simulink model "MOBATSim"  (R2020b)
settings: Solver=FixedStepAuto  StartTime=0.0  StopTime=Sim_t  FixedStep=0.01  MinStep=0.01  RelTol=1e-2
values from neighbouring files (symbols this model uses):
  Vehicles = evalin('base','Vehicles')    [I2V.m]    (also in VehicleSensors.m)
undefined symbols (not defined in the file or in its folder): Sim_Ts
libraries: simulink x50, robotalgslib x10, drivingvehiclecontroller x10, mpcadaslib x10, pid_lib x10
(part 1 of 7)
Description:
  | Main Simulink Model for MOBATSim
settings Model: VariantFading=off  Creator=Mustafa  LastModifiedBy=mustafa
settings SolverCC: AutoInsertRateTranBlk=on  InsertRTBMode=Always  MinimalZcImpactIntegration=on
settings DataIOCC: ReturnWorkspaceOutputs=off
settings DebuggingCC: AlgebraicLoopMsg=error  UniqueDataStoreMsg=error  ArithmeticOperatorsInVariantConditions=warning
settings SFSimCC: SimUseLocalCustomCode=off  CustomCodeUndefinedFunction=UseInterfaceOnly
settings RTWCC: RTWUseLocalCustomCode=off
settings CodeAppCC: StateflowObjectComments=on

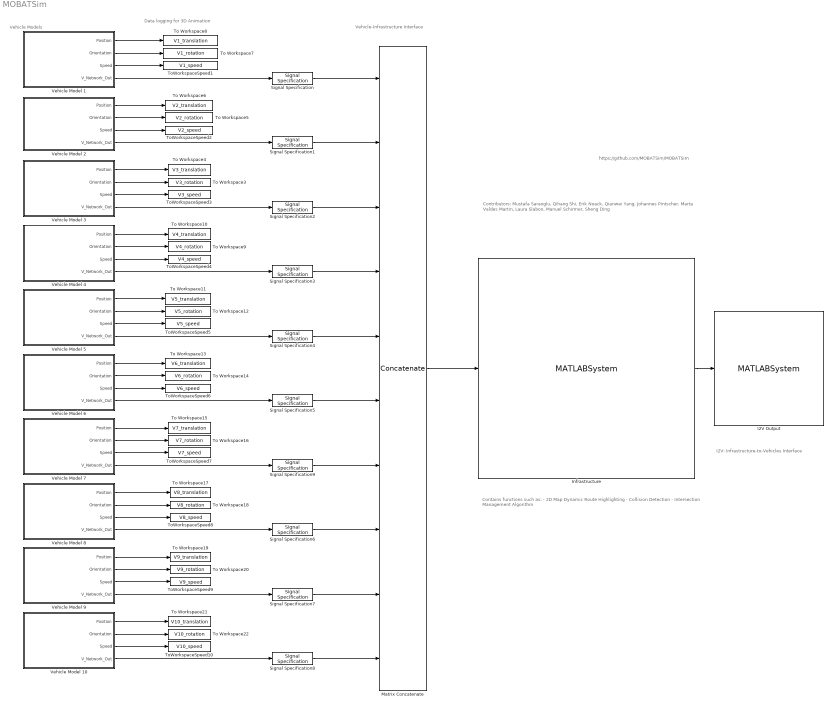
== system MOBATSim ==
  note: Contributors: Mustafa Saraoglu, Qihang Shi, Erik Noack, Qianwei Yang, Johannes Pintscher, Marta Valdes Martin, Laura Slabon, Manuel Schirmer, Sheng Ding
  note: https://github.com/MOBATSim/MOBATSim
  note: Data logging for 3D Animation
  note: Vehicle Models
  note: Vehicle-Infrastructure Interface
  note: I2V: Infrastructure-to-Vehicles Interface
  note: Contains functions such as:
      | - 2D Map Dynamic Route Highlighting
      | - Collision Detection
      | - Intersection Management Algorithm
  I2V Output : MATLABSystem  System=I2V  SimulateUsing=Interpreted execution
      mask Type: I2V
      mask Display:
      | image('MOBATSIM-Icon-Set_3- Flags.png');
      | port_label('input',1,'Flags');
  Infrastructure : MATLABSystem  Description=An instance of the Map.m Class is created.  System=Infrastructure  nrVehicles=length(Vehicles)  SimulateUsing=Interpreted execution
      mask Type: Infrastructure
      mask Display:
      | image('MOBATSIM-Icon-Set_5- Intersection.png');
      | port_label('input',1,'V2Idata');
      | port_label('output',1,'StopCommands');
  Matrix Concatenate : Concatenate  NumInputs=10  Mode=Multidimensional array
  Signal Specification{,1..9} (10 alike) : SignalSpecification  Dimensions=[1 2]
  To Workspace10 : ToWorkspace  VariableName=V4_translation  SaveFormat=Timeseries  SampleTime=-1
  To Workspace11 : ToWorkspace  VariableName=V5_translation  SaveFormat=Timeseries  SampleTime=-1
  To Workspace12 : ToWorkspace  VariableName=V5_rotation  SaveFormat=Timeseries  SampleTime=-1
  To Workspace13 : ToWorkspace  VariableName=V6_translation  SaveFormat=Timeseries  SampleTime=-1
  To Workspace14 : ToWorkspace  VariableName=V6_rotation  SaveFormat=Timeseries  SampleTime=-1
  To Workspace15 : ToWorkspace  VariableName=V7_translation  SaveFormat=Timeseries  SampleTime=-1
  To Workspace16 : ToWorkspace  VariableName=V7_rotation  SaveFormat=Timeseries  SampleTime=-1
  To Workspace17 : ToWorkspace  VariableName=V8_translation  SaveFormat=Timeseries  SampleTime=-1
  To Workspace18 : ToWorkspace  VariableName=V8_rotation  SaveFormat=Timeseries  SampleTime=-1
  To Workspace19 : ToWorkspace  VariableName=V9_translation  SaveFormat=Timeseries  SampleTime=-1
  To Workspace20 : ToWorkspace  VariableName=V9_rotation  SaveFormat=Timeseries  SampleTime=-1
  To Workspace21 : ToWorkspace  VariableName=V10_translation  SaveFormat=Timeseries  SampleTime=-1
  To Workspace22 : ToWorkspace  VariableName=V10_rotation  SaveFormat=Timeseries  SampleTime=-1
  To Workspace3 : ToWorkspace  VariableName=V3_rotation  SaveFormat=Timeseries  SampleTime=-1
  To Workspace4 : ToWorkspace  VariableName=V3_translation  SaveFormat=Timeseries  SampleTime=-1
  To Workspace5 : ToWorkspace  VariableName=V2_rotation  SaveFormat=Timeseries  SampleTime=-1
  To Workspace6 : ToWorkspace  VariableName=V2_translation  SaveFormat=Timeseries  SampleTime=-1
  To Workspace7 : ToWorkspace  VariableName=V1_rotation  SaveFormat=Timeseries  SampleTime=-1
  To Workspace8 : ToWorkspace  VariableName=V1_translation  SaveFormat=Timeseries  SampleTime=-1
  To Workspace9 : ToWorkspace  VariableName=V4_rotation  SaveFormat=Timeseries  SampleTime=-1
  ToWorkspaceSpeed1 : ToWorkspace  VariableName=V1_speed  SaveFormat=Timeseries  SampleTime=-1
  ToWorkspaceSpeed10 : ToWorkspace  VariableName=V10_speed  SaveFormat=Timeseries  SampleTime=-1
  ToWorkspaceSpeed2 : ToWorkspace  VariableName=V2_speed  SaveFormat=Timeseries  SampleTime=-1
  "ToWorkspaceSpeed3 " : ToWorkspace  VariableName=V3_speed  SaveFormat=Timeseries  SampleTime=-1
  ToWorkspaceSpeed4 : ToWorkspace  VariableName=V4_speed  SaveFormat=Timeseries  SampleTime=-1
  ToWorkspaceSpeed5 : ToWorkspace  VariableName=V5_speed  SaveFormat=Timeseries  SampleTime=-1
  ToWorkspaceSpeed6 : ToWorkspace  VariableName=V6_speed  SaveFormat=Timeseries  SampleTime=-1
  ToWorkspaceSpeed7 : ToWorkspace  VariableName=V7_speed  SaveFormat=Timeseries  SampleTime=-1
  ToWorkspaceSpeed8 : ToWorkspace  VariableName=V8_speed  SaveFormat=Timeseries  SampleTime=-1
  ToWorkspaceSpeed9 : ToWorkspace  VariableName=V9_speed  SaveFormat=Timeseries  SampleTime=-1
  Vehicle Model 1 : Subsystem  Description=Tag: Autonomous Vehicle Model  SystemSampleTime=0.01  mask{Vehicle_id=1}
      mask TypeOptions Vehicle_id: MATLAB System2/Vehicle_id
      mask DialogControl DescTextVar Prompt: Autonomous Vehicle Model defined as a system, press the arrow on the lower left corner to see the subsystems. The initial parameters below should be taken from the base workspace but you can edit them anyway you like.
      mask Display: image('$imagefile'); % Use "Edit Image" on toolstrip to change.
  Vehicle Model 10 : Subsystem  Description=Tag: Autonomous Vehicle Model  SystemSampleTime=0.01  mask{Vehicle_id=10}
      mask TypeOptions Vehicle_id: MATLAB System2/Vehicle_id
      mask DialogControl DescTextVar Prompt: Autonomous Vehicle Model defined as a system, press the arrow on the lower left corner to see the subsystems. The initial parameters below should be taken from the base workspace but you can edit them anyway you like.
      mask Display: image('$imagefile'); % Use "Edit Image" on toolstrip to change.
  Vehicle Model 2 : Subsystem  Description=Tag: Autonomous Vehicle Model  SystemSampleTime=0.01  mask{Vehicle_id=2}
      mask TypeOptions Vehicle_id: MATLAB System2/Vehicle_id
      mask DialogControl DescTextVar Prompt: Autonomous Vehicle Model defined as a system, press the arrow on the lower left corner to see the subsystems. The initial parameters below should be taken from the base workspace but you can edit them anyway you like.
      mask Display: image('$imagefile'); % Use "Edit Image" on toolstrip to change.
  Vehicle Model 3 : Subsystem  Description=Tag: Autonomous Vehicle Model  SystemSampleTime=0.01  mask{Vehicle_id=3}
      mask TypeOptions Vehicle_id: MATLAB System2/Vehicle_id
      mask DialogControl DescTextVar Prompt: Autonomous Vehicle Model defined as a system, press the arrow on the lower left corner to see the subsystems. The initial parameters below should be taken from the base workspace but you can edit them anyway you like.
      mask Display: image('$imagefile'); % Use "Edit Image" on toolstrip to change.
  Vehicle Model 4 : Subsystem  Description=Tag: Autonomous Vehicle Model  SystemSampleTime=0.01  mask{Vehicle_id=4}
      mask TypeOptions Vehicle_id: MATLAB System2/Vehicle_id
      mask DialogControl DescTextVar Prompt: Autonomous Vehicle Model defined as a system, press the arrow on the lower left corner to see the subsystems. The initial parameters below should be taken from the base workspace but you can edit them anyway you like.
      mask Display: image('$imagefile'); % Use "Edit Image" on toolstrip to change.
  Vehicle Model 5 : Subsystem  Description=Tag: Autonomous Vehicle Model  SystemSampleTime=0.01  mask{Vehicle_id=5}
      mask TypeOptions Vehicle_id: MATLAB System2/Vehicle_id
      mask DialogControl DescTextVar Prompt: Autonomous Vehicle Model defined as a system, press the arrow on the lower left corner to see the subsystems. The initial parameters below should be taken from the base workspace but you can edit them anyway you like.
      mask Display: image('$imagefile'); % Use "Edit Image" on toolstrip to change.
  Vehicle Model 6 : Subsystem  Description=Tag: Autonomous Vehicle Model  SystemSampleTime=0.01  mask{Vehicle_id=6}
      mask TypeOptions Vehicle_id: MATLAB System2/Vehicle_id
      mask DialogControl DescTextVar Prompt: Autonomous Vehicle Model defined as a system, press the arrow on the lower left corner to see the subsystems. The initial parameters below should be taken from the base workspace but you can edit them anyway you like.
      mask Display: image('$imagefile'); % Use "Edit Image" on toolstrip to change.
  Vehicle Model 7 : Subsystem  Description=Tag: Autonomous Vehicle Model  SystemSampleTime=0.01  mask{Vehicle_id=7}
      mask TypeOptions Vehicle_id: MATLAB System2/Vehicle_id
      mask DialogControl DescTextVar Prompt: Autonomous Vehicle Model defined as a system, press the arrow on the lower left corner to see the subsystems. The initial parameters below should be taken from the base workspace but you can edit them anyway you like.
      mask Display: image('$imagefile'); % Use "Edit Image" on toolstrip to change.
  Vehicle Model 8 : Subsystem  Description=Tag: Autonomous Vehicle Model  SystemSampleTime=0.01  mask{Vehicle_id=8}
      mask TypeOptions Vehicle_id: MATLAB System2/Vehicle_id
      mask DialogControl DescTextVar Prompt: Autonomous Vehicle Model defined as a system, press the arrow on the lower left corner to see the subsystems. The initial parameters below should be taken from the base workspace but you can edit them anyway you like.
      mask Display: image('$imagefile'); % Use "Edit Image" on toolstrip to change.
  Vehicle Model 9 : Subsystem  Description=Tag: Autonomous Vehicle Model  SystemSampleTime=0.01  mask{Vehicle_id=9}
      mask TypeOptions Vehicle_id: MATLAB System2/Vehicle_id
      mask DialogControl DescTextVar Prompt: Autonomous Vehicle Model defined as a system, press the arrow on the lower left corner to see the subsystems. The initial parameters below should be taken from the base workspace but you can edit them anyway you like.
      mask Display: image('$imagefile'); % Use "Edit Image" on toolstrip to change.
  wires:
  Vehicle Model 1/1(Position) -> To Workspace8/1
  Vehicle Model 1/2(Orientation) -> To Workspace7/1
  Vehicle Model 1/4(V_Network_Out) -> Signal Specification/1
  Signal Specification/1 -> Matrix Concatenate/1
  Signal Specification1/1 -> Matrix Concatenate/2
  Vehicle Model 2/2(Orientation) -> To Workspace5/1
  Vehicle Model 2/1(Position) -> To Workspace6/1
  Vehicle Model 3/2(Orientation) -> To Workspace3/1
  Vehicle Model 3/1(Position) -> To Workspace4/1
  Signal Specification2/1 -> Matrix Concatenate/3
  Infrastructure/1 -> I2V Output/1
  Vehicle Model 8/4(V_Network_Out) -> Signal Specification6/1
  Vehicle Model 9/4(V_Network_Out) -> Signal Specification7/1
  Vehicle Model 10/4(V_Network_Out) -> Signal Specification8/1
  Signal Specification3/1 -> Matrix Concatenate/4
  Signal Specification4/1 -> Matrix Concatenate/5
  Signal Specification5/1 -> Matrix Concatenate/6
  Signal Specification9/1 -> Matrix Concatenate/7
  Signal Specification6/1 -> Matrix Concatenate/8
  Signal Specification7/1 -> Matrix Concatenate/9
  Signal Specification8/1 -> Matrix Concatenate/10
  Vehicle Model 4/2(Orientation) -> To Workspace9/1
  Vehicle Model 4/1(Position) -> To Workspace10/1
  Vehicle Model 6/2(Orientation) -> To Workspace14/1
  Vehicle Model 6/1(Position) -> To Workspace13/1
  Vehicle Model 7/2(Orientation) -> To Workspace16/1
  Vehicle Model 7/1(Position) -> To Workspace15/1
  Vehicle Model 8/2(Orientation) -> To Workspace18/1
  Vehicle Model 8/1(Position) -> To Workspace17/1
  Vehicle Model 9/2(Orientation) -> To Workspace20/1
  Vehicle Model 9/1(Position) -> To Workspace19/1
  Vehicle Model 10/2(Orientation) -> To Workspace22/1
  Vehicle Model 10/1(Position) -> To Workspace21/1
  Matrix Concatenate/1 -> Infrastructure/1
  Vehicle Model 2/4(V_Network_Out) -> Signal Specification1/1
  Vehicle Model 3/4(V_Network_Out) -> Signal Specification2/1
  Vehicle Model 4/4(V_Network_Out) -> Signal Specification3/1
  Vehicle Model 6/4(V_Network_Out) -> Signal Specification5/1
  Vehicle Model 7/4(V_Network_Out) -> Signal Specification9/1
  Vehicle Model 5/1(Position) -> To Workspace11/1
  Vehicle Model 5/2(Orientation) -> To Workspace12/1
  Vehicle Model 5/4(V_Network_Out) -> Signal Specification4/1
  Vehicle Model 1/3(Speed) -> ToWorkspaceSpeed1/1
  Vehicle Model 2/3(Speed) -> ToWorkspaceSpeed2/1
  Vehicle Model 3/3(Speed) -> "ToWorkspaceSpeed3 "/1
  Vehicle Model 4/3(Speed) -> ToWorkspaceSpeed4/1
  Vehicle Model 5/3(Speed) -> ToWorkspaceSpeed5/1
  Vehicle Model 6/3(Speed) -> ToWorkspaceSpeed6/1
  Vehicle Model 7/3(Speed) -> ToWorkspaceSpeed7/1
  Vehicle Model 8/3(Speed) -> ToWorkspaceSpeed8/1
  Vehicle Model 9/3(Speed) -> ToWorkspaceSpeed9/1
  Vehicle Model 10/3(Speed) -> ToWorkspaceSpeed10/1

== system MOBATSim/Vehicle Model 1 ==
  note: Perception
  note: Decision-Making
  note: Control
  Behavioural Planner : MATLABSystem  System=VehicleDrivingMode  Vehicle_id=Vehicle_id  SimulateUsing=Interpreted execution
      mask Type: VehicleDrivingMode
      mask Display:
      | image('MOBATSIM-Icon-Set_7- Behavioural Planner.png');
      | port_label('input',1,'vehicleDetected');
      | port_label('output',1,'SpeedReference');
      | port_label('output',2,'DistanceReference');
      | port_label('output',3,'LeadSpeed');
      | port_label('output',4,'DrivingMode');
      | port_label('output',5,'Dist2Stop');
      | port_label('output',6,'laneChange');
  Longitudinal and Lateral Controllers : Subsystem
  Path Planner : Subsystem  Variant=on  VariantControlMode=label  LabelModeActiveChoice=Astar  mask{PathPlanningAlgorithm=Astar}
      mask prompts: PathPlanningAlgorithm "Path Planning Algorithm"
      mask TypeOptions PathPlanningAlgorithm: Astar | ShortestPathFinder
      mask Callback PathPlanningAlgorithm: set_param(gcb,'OverrideUsingVariant',get_param(gcb,'PathPlanningAlgorithm'));
      mask Display: image("MOBATSIM-Icon-Set_8- Navigation.png");
  Transform to MOBATSim Coordinates : Subsystem
  Vehicle Model : Subsystem  mask{Vehicle_id=Vehicle_id}
      mask prompts: Vehicle_id "Vehicle ID"
      mask Display: image('MOBATSIM-Icon-Set_13- VehicleModel.png'); % Use "Edit Image" on toolstrip to change.
  Vehicle Sensors : MATLABSystem  System=VehicleSensors  Vehicle_id=Vehicle_id  Tsample=Sim_Ts  OffsetTime=0  SimulateUsing=Interpreted execution
      mask Type: VehicleSensors
      mask Display:
      | image('MOBATSIM-Icon-Set_4- Sensor.png');
      | port_label('output',1,'V2VcommIDs');
      | port_label('output',2,'vehicleDetected');
  Vehicle Status Check and Acceleration to Speed : Subsystem
  Vehicle V2I Output : MATLABSystem  System=VehicleV2I_Out  Vehicle_id=Vehicle_id  SimulateUsing=Interpreted execution
      mask Type: VehicleV2I_Out
      mask Display:
      | image('MOBATSIM-Icon-Set_6- V2l.png');
      | port_label('input',1,'waypointReached');
      | port_label('output',1,'V2Idata');
  Position : Outport  VectorParamsAs1DForOutWhenUnconnected=off
  Orientation : Outport  Port=2  VectorParamsAs1DForOutWhenUnconnected=off
  Speed : Outport  Port=3  VectorParamsAs1DForOutWhenUnconnected=off
  V_Network_Out : Outport  Port=4  VectorParamsAs1DForOutWhenUnconnected=off
  wires:
  Vehicle V2I Output/1 -> V_Network_Out/1
  Vehicle Sensors/2 -> Behavioural Planner/1
  Behavioural Planner/1 -> Longitudinal and Lateral Controllers/1(Speed Reference)
  Behavioural Planner/2 -> Longitudinal and Lateral Controllers/2(Inter Vehicular Distance)
  Behavioural Planner/3 -> Longitudinal and Lateral Controllers/3(Lead Speed)
  Behavioural Planner/4 -> Longitudinal and Lateral Controllers/4(drivingMode)
  Behavioural Planner/5 -> Longitudinal and Lateral Controllers/5(Dist2Stop)
  Transform to MOBATSim Coordinates/1(Position) -> Position/1
  Transform to MOBATSim Coordinates/2(Orientation) -> Orientation/1
  Vehicle Model/2(Speed) -> Longitudinal and Lateral Controllers/8(Actual Speed), Speed/1
  Vehicle Model/1(Pose) -> Longitudinal and Lateral Controllers/7(Actual Pose), Transform to MOBATSim Coordinates/1(Pose)
  Longitudinal and Lateral Controllers/1(Longitudinal Acceleration Cmd) -> Vehicle Status Check and Acceleration to Speed/1(Reference Acceleration)
  Longitudinal and Lateral Controllers/2(Reference Steering Angle) -> Vehicle Status Check and Acceleration to Speed/2(Reference Steering Angle)
  Vehicle Status Check and Acceleration to Speed/2(Steering Angle Cmd) -> Vehicle Model/2(Steering Angle)
  Behavioural Planner/6 -> Longitudinal and Lateral Controllers/6(laneChange)
  Vehicle Sensors/1 -> Path Planner/1(CommunicationIDs)
  Path Planner/1(waypointReached) -> Vehicle V2I Output/1
  Vehicle Status Check and Acceleration to Speed/1(Speed Cmd) -> Vehicle Model/1(Longitudinal Speed)

== system MOBATSim/Vehicle Model 10 ==
  note: Perception
  note: Decision-Making
  note: Control
  Behavioural Planner : MATLABSystem  System=VehicleDrivingMode  Vehicle_id=Vehicle_id  SimulateUsing=Interpreted execution
      mask Type: VehicleDrivingMode
      mask Display:
      | image('MOBATSIM-Icon-Set_7- Behavioural Planner.png');
      | port_label('input',1,'vehicleDetected');
      | port_label('output',1,'SpeedReference');
      | port_label('output',2,'DistanceReference');
      | port_label('output',3,'LeadSpeed');
      | port_label('output',4,'DrivingMode');
      | port_label('output',5,'Dist2Stop');
      | port_label('output',6,'laneChange');
  Longitudinal and Lateral Controllers : Subsystem
  Path Planner : Subsystem  Variant=on  VariantControlMode=label  LabelModeActiveChoice=Astar  mask{PathPlanningAlgorithm=Astar}
      mask prompts: PathPlanningAlgorithm "Path Planning Algorithm"
      mask TypeOptions PathPlanningAlgorithm: Astar | ShortestPathFinder
      mask Callback PathPlanningAlgorithm: set_param(gcb,'OverrideUsingVariant',get_param(gcb,'PathPlanningAlgorithm'));
      mask Display: image("MOBATSIM-Icon-Set_8- Navigation.png");
  Transform to MOBATSim Coordinates : Subsystem
  Vehicle Model : Subsystem  mask{Vehicle_id=Vehicle_id}
      mask prompts: Vehicle_id "Vehicle ID"
      mask Display: image('MOBATSIM-Icon-Set_13- VehicleModel.png'); % Use "Edit Image" on toolstrip to change.
  Vehicle Sensors : MATLABSystem  System=VehicleSensors  Vehicle_id=Vehicle_id  Tsample=Sim_Ts  OffsetTime=0  SimulateUsing=Interpreted execution
      mask Type: VehicleSensors
      mask Display:
      | image('MOBATSIM-Icon-Set_4- Sensor.png');
      | port_label('output',1,'V2VcommIDs');
      | port_label('output',2,'vehicleDetected');
  Vehicle Status Check and Acceleration to Speed : Subsystem
  Vehicle V2I Output : MATLABSystem  System=VehicleV2I_Out  Vehicle_id=Vehicle_id  SimulateUsing=Interpreted execution
      mask Type: VehicleV2I_Out
      mask Display:
      | image('MOBATSIM-Icon-Set_6- V2l.png');
      | port_label('input',1,'waypointReached');
      | port_label('output',1,'V2Idata');
  Position : Outport  VectorParamsAs1DForOutWhenUnconnected=off
  Orientation : Outport  Port=2  VectorParamsAs1DForOutWhenUnconnected=off
  Speed : Outport  Port=3  VectorParamsAs1DForOutWhenUnconnected=off
  V_Network_Out : Outport  Port=4  VectorParamsAs1DForOutWhenUnconnected=off
  wires:
  Vehicle V2I Output/1 -> V_Network_Out/1
  Vehicle Sensors/2 -> Behavioural Planner/1
  Behavioural Planner/1 -> Longitudinal and Lateral Controllers/1(Speed Reference)
  Behavioural Planner/2 -> Longitudinal and Lateral Controllers/2(Inter Vehicular Distance)
  Behavioural Planner/3 -> Longitudinal and Lateral Controllers/3(Lead Speed)
  Behavioural Planner/4 -> Longitudinal and Lateral Controllers/4(drivingMode)
  Behavioural Planner/5 -> Longitudinal and Lateral Controllers/5(Dist2Stop)
  Transform to MOBATSim Coordinates/1(Position) -> Position/1
  Transform to MOBATSim Coordinates/2(Orientation) -> Orientation/1
  Vehicle Model/2(Speed) -> Longitudinal and Lateral Controllers/8(Actual Speed), Speed/1
  Vehicle Model/1(Pose) -> Longitudinal and Lateral Controllers/7(Actual Pose), Transform to MOBATSim Coordinates/1(Pose)
  Longitudinal and Lateral Controllers/1(Longitudinal Acceleration Cmd) -> Vehicle Status Check and Acceleration to Speed/1(Reference Acceleration)
  Longitudinal and Lateral Controllers/2(Reference Steering Angle) -> Vehicle Status Check and Acceleration to Speed/2(Reference Steering Angle)
  Vehicle Status Check and Acceleration to Speed/2(Steering Angle Cmd) -> Vehicle Model/2(Steering Angle)
  Behavioural Planner/6 -> Longitudinal and Lateral Controllers/6(laneChange)
  Vehicle Sensors/1 -> Path Planner/1(CommunicationIDs)
  Path Planner/1(waypointReached) -> Vehicle V2I Output/1
  Vehicle Status Check and Acceleration to Speed/1(Speed Cmd) -> Vehicle Model/1(Longitudinal Speed)

== system MOBATSim/Vehicle Model 2 ==
  note: Decision-Making
  note: Control
  note: Perception
  note: Vehicle 2: Ego Vehicle in 3D
      | - Lane-changing on double-lane routes
  Behavioural Planner - Ego Vehicle : MATLABSystem  System=VehicleDrivingMode_Ego  Vehicle_id=Vehicle_id  SimulateUsing=Interpreted execution
      mask Type: VehicleDrivingMode_Ego
      mask Display:
      | image('MOBATSIM-Icon-Set_7- Behavioural Planner.png');
      | port_label('input',1,'vehicleDetected');
      | port_label('output',1,'SpeedReference');
      | port_label('output',2,'DistanceReference');
      | port_label('output',3,'LeadSpeed');
      | port_label('output',4,'DrivingMode');
      | port_label('output',5,'Dist2Stop');
      | port_label('output',6,'laneChange');
  Longitudinal and Lateral Controllers : Subsystem
  Path Planner : Subsystem  Variant=on  VariantControlMode=label  LabelModeActiveChoice=Astar  mask{PathPlanningAlgorithm=Astar}
      mask prompts: PathPlanningAlgorithm "Path Planning Algorithm"
      mask TypeOptions PathPlanningAlgorithm: Astar | ShortestPathFinder
      mask Callback PathPlanningAlgorithm: set_param(gcb,'OverrideUsingVariant',get_param(gcb,'PathPlanningAlgorithm'));
      mask Display: image("MOBATSIM-Icon-Set_8- Navigation.png");
  Transform to MOBATSim Coordinates : Subsystem
  Vehicle Model : Subsystem  mask{Vehicle_id=Vehicle_id}
      mask prompts: Vehicle_id "Vehicle ID"
      mask Display: image('MOBATSIM-Icon-Set_13- VehicleModel.png'); % Use "Edit Image" on toolstrip to change.
  Vehicle Sensors : MATLABSystem  System=VehicleSensors  Vehicle_id=Vehicle_id  Tsample=Sim_Ts  OffsetTime=0  SimulateUsing=Interpreted execution
      mask Type: VehicleSensors
      mask Display:
      | image('MOBATSIM-Icon-Set_4- Sensor.png');
      | port_label('output',1,'V2VcommIDs');
      | port_label('output',2,'vehicleDetected');
  Vehicle Status Check and Acceleration to Speed : Subsystem
  Vehicle V2I Output : MATLABSystem  System=VehicleV2I_Out  Vehicle_id=Vehicle_id  SimulateUsing=Interpreted execution
      mask Type: VehicleV2I_Out
      mask Display:
      | image('MOBATSIM-Icon-Set_6- V2l.png');
      | port_label('input',1,'waypointReached');
      | port_label('output',1,'V2Idata');
  Position : Outport  VectorParamsAs1DForOutWhenUnconnected=off
  Orientation : Outport  Port=2  VectorParamsAs1DForOutWhenUnconnected=off
  Speed : Outport  Port=3  VectorParamsAs1DForOutWhenUnconnected=off
  V_Network_Out : Outport  Port=4  VectorParamsAs1DForOutWhenUnconnected=off
  wires:
  Path Planner/1(waypointReached) -> Vehicle V2I Output/1
  Vehicle V2I Output/1 -> V_Network_Out/1
  Transform to MOBATSim Coordinates/1(Position) -> Position/1
  Transform to MOBATSim Coordinates/2(Orientation) -> Orientation/1
  Behavioural Planner - Ego Vehicle/1 -> Longitudinal and Lateral Controllers/1(Speed Reference)
  Behavioural Planner - Ego Vehicle/2 -> Longitudinal and Lateral Controllers/2(Inter Vehicular Distance)
  Behavioural Planner - Ego Vehicle/3 -> Longitudinal and Lateral Controllers/3(Lead Speed)
  Behavioural Planner - Ego Vehicle/4 -> Longitudinal and Lateral Controllers/4(Driving Mode)
  Behavioural Planner - Ego Vehicle/5 -> Longitudinal and Lateral Controllers/5(Dist2Stop)
  Behavioural Planner - Ego Vehicle/6 -> Longitudinal and Lateral Controllers/6(laneChange)
  Vehicle Model/2(Speed) -> Speed/1, Longitudinal and Lateral Controllers/8(Actual Speed)
  Vehicle Model/1(Pose) -> Transform to MOBATSim Coordinates/1(Pose), Longitudinal and Lateral Controllers/7(Actual Pose)
  Longitudinal and Lateral Controllers/1(Longitudinal Acceleration Cmd) -> Vehicle Status Check and Acceleration to Speed/1(Reference Acceleration)
  Longitudinal and Lateral Controllers/2(Reference Steering Angle) -> Vehicle Status Check and Acceleration to Speed/2(Reference Steering Angle)
  Vehicle Status Check and Acceleration to Speed/2(Steering Angle Cmd) -> Vehicle Model/2(Steering Angle)
  Vehicle Status Check and Acceleration to Speed/1(Speed Cmd) -> Vehicle Model/1(Longitudinal Speed)
  Vehicle Sensors/2 -> Behavioural Planner - Ego Vehicle/1
  Vehicle Sensors/1 -> Path Planner/1(CommunicationIDs)

== system MOBATSim/Vehicle Model 3 ==
  note: Perception
  note: Decision-Making
  note: Control
  Behavioural Planner : MATLABSystem  System=VehicleDrivingMode  Vehicle_id=Vehicle_id  SimulateUsing=Interpreted execution
      mask Type: VehicleDrivingMode
      mask Display:
      | image('MOBATSIM-Icon-Set_7- Behavioural Planner.png');
      | port_label('input',1,'vehicleDetected');
      | port_label('output',1,'SpeedReference');
      | port_label('output',2,'DistanceReference');
      | port_label('output',3,'LeadSpeed');
      | port_label('output',4,'DrivingMode');
      | port_label('output',5,'Dist2Stop');
      | port_label('output',6,'laneChange');
  Longitudinal and Lateral Controllers : Subsystem
  Path Planner : Subsystem  Variant=on  VariantControlMode=label  LabelModeActiveChoice=Astar  mask{PathPlanningAlgorithm=Astar}
      mask prompts: PathPlanningAlgorithm "Path Planning Algorithm"
      mask TypeOptions PathPlanningAlgorithm: Astar | ShortestPathFinder
      mask Callback PathPlanningAlgorithm: set_param(gcb,'OverrideUsingVariant',get_param(gcb,'PathPlanningAlgorithm'));
      mask Display: image("MOBATSIM-Icon-Set_8- Navigation.png");
  Transform to MOBATSim Coordinates : Subsystem
  Vehicle Model : Subsystem  mask{Vehicle_id=Vehicle_id}
      mask prompts: Vehicle_id "Vehicle ID"
      mask Display: image('MOBATSIM-Icon-Set_13- VehicleModel.png'); % Use "Edit Image" on toolstrip to change.
  Vehicle Sensors : MATLABSystem  System=VehicleSensors  Vehicle_id=Vehicle_id  Tsample=Sim_Ts  OffsetTime=0  SimulateUsing=Interpreted execution
      mask Type: VehicleSensors
      mask Display:
      | image('MOBATSIM-Icon-Set_4- Sensor.png');
      | port_label('output',1,'V2VcommIDs');
      | port_label('output',2,'vehicleDetected');
  Vehicle Status Check and Acceleration to Speed : Subsystem
  Vehicle V2I Output : MATLABSystem  System=VehicleV2I_Out  Vehicle_id=Vehicle_id  SimulateUsing=Interpreted execution
      mask Type: VehicleV2I_Out
      mask Display:
      | image('MOBATSIM-Icon-Set_6- V2l.png');
      | port_label('input',1,'waypointReached');
      | port_label('output',1,'V2Idata');
  Position : Outport  VectorParamsAs1DForOutWhenUnconnected=off
  Orientation : Outport  Port=2  VectorParamsAs1DForOutWhenUnconnected=off
  Speed : Outport  Port=3  VectorParamsAs1DForOutWhenUnconnected=off
  V_Network_Out : Outport  Port=4  VectorParamsAs1DForOutWhenUnconnected=off
  wires:
  Vehicle V2I Output/1 -> V_Network_Out/1
  Vehicle Sensors/2 -> Behavioural Planner/1
  Behavioural Planner/1 -> Longitudinal and Lateral Controllers/1(Speed Reference)
  Behavioural Planner/2 -> Longitudinal and Lateral Controllers/2(Inter Vehicular Distance)
  Behavioural Planner/3 -> Longitudinal and Lateral Controllers/3(Lead Speed)
  Behavioural Planner/4 -> Longitudinal and Lateral Controllers/4(drivingMode)
  Behavioural Planner/5 -> Longitudinal and Lateral Controllers/5(Dist2Stop)
  Transform to MOBATSim Coordinates/1(Position) -> Position/1
  Transform to MOBATSim Coordinates/2(Orientation) -> Orientation/1
  Vehicle Model/2(Speed) -> Longitudinal and Lateral Controllers/8(Actual Speed), Speed/1
  Vehicle Model/1(Pose) -> Longitudinal and Lateral Controllers/7(Actual Pose), Transform to MOBATSim Coordinates/1(Pose)
  Longitudinal and Lateral Controllers/1(Longitudinal Acceleration Cmd) -> Vehicle Status Check and Acceleration to Speed/1(Reference Acceleration)
  Longitudinal and Lateral Controllers/2(Reference Steering Angle) -> Vehicle Status Check and Acceleration to Speed/2(Reference Steering Angle)
  Vehicle Status Check and Acceleration to Speed/2(Steering Angle Cmd) -> Vehicle Model/2(Steering Angle)
  Behavioural Planner/6 -> Longitudinal and Lateral Controllers/6(laneChange)
  Vehicle Sensors/1 -> Path Planner/1(CommunicationIDs)
  Path Planner/1(waypointReached) -> Vehicle V2I Output/1
  Vehicle Status Check and Acceleration to Speed/1(Speed Cmd) -> Vehicle Model/1(Longitudinal Speed)

== system MOBATSim/Vehicle Model 4 ==
  note: Perception
  note: Decision-Making
  note: Control
  Behavioural Planner : MATLABSystem  System=VehicleDrivingMode  Vehicle_id=Vehicle_id  SimulateUsing=Interpreted execution
      mask Type: VehicleDrivingMode
      mask Display:
      | image('MOBATSIM-Icon-Set_7- Behavioural Planner.png');
      | port_label('input',1,'vehicleDetected');
      | port_label('output',1,'SpeedReference');
      | port_label('output',2,'DistanceReference');
      | port_label('output',3,'LeadSpeed');
      | port_label('output',4,'DrivingMode');
      | port_label('output',5,'Dist2Stop');
      | port_label('output',6,'laneChange');
  Longitudinal and Lateral Controllers : Subsystem
  Path Planner : Subsystem  Variant=on  VariantControlMode=label  LabelModeActiveChoice=Astar  mask{PathPlanningAlgorithm=Astar}
      mask prompts: PathPlanningAlgorithm "Path Planning Algorithm"
      mask TypeOptions PathPlanningAlgorithm: Astar | ShortestPathFinder
      mask Callback PathPlanningAlgorithm: set_param(gcb,'OverrideUsingVariant',get_param(gcb,'PathPlanningAlgorithm'));
      mask Display: image("MOBATSIM-Icon-Set_8- Navigation.png");
  Transform to MOBATSim Coordinates : Subsystem
  Vehicle Model : Subsystem  mask{Vehicle_id=Vehicle_id}
      mask prompts: Vehicle_id "Vehicle ID"
      mask Display: image('MOBATSIM-Icon-Set_13- VehicleModel.png'); % Use "Edit Image" on toolstrip to change.
  Vehicle Sensors : MATLABSystem  System=VehicleSensors  Vehicle_id=Vehicle_id  Tsample=Sim_Ts  OffsetTime=0  SimulateUsing=Interpreted execution
      mask Type: VehicleSensors
      mask Display:
      | image('MOBATSIM-Icon-Set_4- Sensor.png');
      | port_label('output',1,'V2VcommIDs');
      | port_label('output',2,'vehicleDetected');
  Vehicle Status Check and Acceleration to Speed : Subsystem
  Vehicle V2I Output : MATLABSystem  System=VehicleV2I_Out  Vehicle_id=Vehicle_id  SimulateUsing=Interpreted execution
      mask Type: VehicleV2I_Out
      mask Display:
      | image('MOBATSIM-Icon-Set_6- V2l.png');
      | port_label('input',1,'waypointReached');
      | port_label('output',1,'V2Idata');
  Position : Outport  VectorParamsAs1DForOutWhenUnconnected=off
  Orientation : Outport  Port=2  VectorParamsAs1DForOutWhenUnconnected=off
  Speed : Outport  Port=3  VectorParamsAs1DForOutWhenUnconnected=off
  V_Network_Out : Outport  Port=4  VectorParamsAs1DForOutWhenUnconnected=off
  wires:
  Vehicle V2I Output/1 -> V_Network_Out/1
  Vehicle Sensors/2 -> Behavioural Planner/1
  Behavioural Planner/1 -> Longitudinal and Lateral Controllers/1(Speed Reference)
  Behavioural Planner/2 -> Longitudinal and Lateral Controllers/2(Inter Vehicular Distance)
  Behavioural Planner/3 -> Longitudinal and Lateral Controllers/3(Lead Speed)
  Behavioural Planner/4 -> Longitudinal and Lateral Controllers/4(drivingMode)
  Behavioural Planner/5 -> Longitudinal and Lateral Controllers/5(Dist2Stop)
  Transform to MOBATSim Coordinates/1(Position) -> Position/1
  Transform to MOBATSim Coordinates/2(Orientation) -> Orientation/1
  Vehicle Model/2(Speed) -> Longitudinal and Lateral Controllers/8(Actual Speed), Speed/1
  Vehicle Model/1(Pose) -> Longitudinal and Lateral Controllers/7(Actual Pose), Transform to MOBATSim Coordinates/1(Pose)
  Longitudinal and Lateral Controllers/1(Longitudinal Acceleration Cmd) -> Vehicle Status Check and Acceleration to Speed/1(Reference Acceleration)
  Longitudinal and Lateral Controllers/2(Reference Steering Angle) -> Vehicle Status Check and Acceleration to Speed/2(Reference Steering Angle)
  Vehicle Status Check and Acceleration to Speed/2(Steering Angle Cmd) -> Vehicle Model/2(Steering Angle)
  Behavioural Planner/6 -> Longitudinal and Lateral Controllers/6(laneChange)
  Vehicle Sensors/1 -> Path Planner/1(CommunicationIDs)
  Path Planner/1(waypointReached) -> Vehicle V2I Output/1
  Vehicle Status Check and Acceleration to Speed/1(Speed Cmd) -> Vehicle Model/1(Longitudinal Speed)

== system MOBATSim/Vehicle Model 5 ==
  note: Perception
  note: Decision-Making
  note: Control
  Behavioural Planner : MATLABSystem  System=VehicleDrivingMode  Vehicle_id=Vehicle_id  SimulateUsing=Interpreted execution
      mask Type: VehicleDrivingMode
      mask Display:
      | image('MOBATSIM-Icon-Set_7- Behavioural Planner.png');
      | port_label('input',1,'vehicleDetected');
      | port_label('output',1,'SpeedReference');
      | port_label('output',2,'DistanceReference');
      | port_label('output',3,'LeadSpeed');
      | port_label('output',4,'DrivingMode');
      | port_label('output',5,'Dist2Stop');
      | port_label('output',6,'laneChange');
  Longitudinal and Lateral Controllers : Subsystem
  Path Planner : Subsystem  Variant=on  VariantControlMode=label  LabelModeActiveChoice=Astar  mask{PathPlanningAlgorithm=Astar}
      mask prompts: PathPlanningAlgorithm "Path Planning Algorithm"
      mask TypeOptions PathPlanningAlgorithm: Astar | ShortestPathFinder
      mask Callback PathPlanningAlgorithm: set_param(gcb,'OverrideUsingVariant',get_param(gcb,'PathPlanningAlgorithm'));
      mask Display: image("MOBATSIM-Icon-Set_8- Navigation.png");
  Transform to MOBATSim Coordinates : Subsystem
  Vehicle Model : Subsystem  mask{Vehicle_id=Vehicle_id}
      mask prompts: Vehicle_id "Vehicle ID"
      mask Display: image('MOBATSIM-Icon-Set_13- VehicleModel.png'); % Use "Edit Image" on toolstrip to change.
  Vehicle Sensors : MATLABSystem  System=VehicleSensors  Vehicle_id=Vehicle_id  Tsample=Sim_Ts  OffsetTime=0  SimulateUsing=Interpreted execution
      mask Type: VehicleSensors
      mask Display:
      | image('MOBATSIM-Icon-Set_4- Sensor.png');
      | port_label('output',1,'V2VcommIDs');
      | port_label('output',2,'vehicleDetected');
  Vehicle Status Check and Acceleration to Speed : Subsystem
  Vehicle V2I Output : MATLABSystem  System=VehicleV2I_Out  Vehicle_id=Vehicle_id  SimulateUsing=Interpreted execution
      mask Type: VehicleV2I_Out
      mask Display:
      | image('MOBATSIM-Icon-Set_6- V2l.png');
      | port_label('input',1,'waypointReached');
      | port_label('output',1,'V2Idata');
  Position : Outport  VectorParamsAs1DForOutWhenUnconnected=off
  Orientation : Outport  Port=2  VectorParamsAs1DForOutWhenUnconnected=off
  Speed : Outport  Port=3  VectorParamsAs1DForOutWhenUnconnected=off
  V_Network_Out : Outport  Port=4  VectorParamsAs1DForOutWhenUnconnected=off
  wires:
  Vehicle V2I Output/1 -> V_Network_Out/1
  Vehicle Sensors/2 -> Behavioural Planner/1
  Behavioural Planner/1 -> Longitudinal and Lateral Controllers/1(Speed Reference)
  Behavioural Planner/2 -> Longitudinal and Lateral Controllers/2(Inter Vehicular Distance)
  Behavioural Planner/3 -> Longitudinal and Lateral Controllers/3(Lead Speed)
  Behavioural Planner/4 -> Longitudinal and Lateral Controllers/4(drivingMode)
  Behavioural Planner/5 -> Longitudinal and Lateral Controllers/5(Dist2Stop)
  Transform to MOBATSim Coordinates/1(Position) -> Position/1
  Transform to MOBATSim Coordinates/2(Orientation) -> Orientation/1
  Vehicle Model/2(Speed) -> Longitudinal and Lateral Controllers/8(Actual Speed), Speed/1
  Vehicle Model/1(Pose) -> Longitudinal and Lateral Controllers/7(Actual Pose), Transform to MOBATSim Coordinates/1(Pose)
  Longitudinal and Lateral Controllers/1(Longitudinal Acceleration Cmd) -> Vehicle Status Check and Acceleration to Speed/1(Reference Acceleration)
  Longitudinal and Lateral Controllers/2(Reference Steering Angle) -> Vehicle Status Check and Acceleration to Speed/2(Reference Steering Angle)
  Vehicle Status Check and Acceleration to Speed/2(Steering Angle Cmd) -> Vehicle Model/2(Steering Angle)
  Behavioural Planner/6 -> Longitudinal and Lateral Controllers/6(laneChange)
  Vehicle Sensors/1 -> Path Planner/1(CommunicationIDs)
  Path Planner/1(waypointReached) -> Vehicle V2I Output/1
  Vehicle Status Check and Acceleration to Speed/1(Speed Cmd) -> Vehicle Model/1(Longitudinal Speed)

== system MOBATSim/Vehicle Model 6 ==
  note: Perception
  note: Decision-Making
  note: Control
  Behavioural Planner : MATLABSystem  System=VehicleDrivingMode  Vehicle_id=Vehicle_id  SimulateUsing=Interpreted execution
      mask Type: VehicleDrivingMode
      mask Display:
      | image('MOBATSIM-Icon-Set_7- Behavioural Planner.png');
      | port_label('input',1,'vehicleDetected');
      | port_label('output',1,'SpeedReference');
      | port_label('output',2,'DistanceReference');
      | port_label('output',3,'LeadSpeed');
      | port_label('output',4,'DrivingMode');
      | port_label('output',5,'Dist2Stop');
      | port_label('output',6,'laneChange');
  Longitudinal and Lateral Controllers : Subsystem
  Path Planner : Subsystem  Variant=on  VariantControlMode=label  LabelModeActiveChoice=Astar  mask{PathPlanningAlgorithm=Astar}
      mask prompts: PathPlanningAlgorithm "Path Planning Algorithm"
      mask TypeOptions PathPlanningAlgorithm: Astar | ShortestPathFinder
      mask Callback PathPlanningAlgorithm: set_param(gcb,'OverrideUsingVariant',get_param(gcb,'PathPlanningAlgorithm'));
      mask Display: image("MOBATSIM-Icon-Set_8- Navigation.png");
  Transform to MOBATSim Coordinates : Subsystem
  Vehicle Model : Subsystem  mask{Vehicle_id=Vehicle_id}
      mask prompts: Vehicle_id "Vehicle ID"
      mask Display: image('MOBATSIM-Icon-Set_13- VehicleModel.png'); % Use "Edit Image" on toolstrip to change.
  Vehicle Sensors : MATLABSystem  System=VehicleSensors  Vehicle_id=Vehicle_id  Tsample=Sim_Ts  OffsetTime=0  SimulateUsing=Interpreted execution
      mask Type: VehicleSensors
      mask Display:
      | image('MOBATSIM-Icon-Set_4- Sensor.png');
      | port_label('output',1,'V2VcommIDs');
      | port_label('output',2,'vehicleDetected');
  Vehicle Status Check and Acceleration to Speed : Subsystem
  Vehicle V2I Output : MATLABSystem  System=VehicleV2I_Out  Vehicle_id=Vehicle_id  SimulateUsing=Interpreted execution
      mask Type: VehicleV2I_Out
      mask Display:
      | image('MOBATSIM-Icon-Set_6- V2l.png');
      | port_label('input',1,'waypointReached');
      | port_label('output',1,'V2Idata');
  Position : Outport  VectorParamsAs1DForOutWhenUnconnected=off
  Orientation : Outport  Port=2  VectorParamsAs1DForOutWhenUnconnected=off
  Speed : Outport  Port=3  VectorParamsAs1DForOutWhenUnconnected=off
  V_Network_Out : Outport  Port=4  VectorParamsAs1DForOutWhenUnconnected=off
  wires:
  Vehicle V2I Output/1 -> V_Network_Out/1
  Vehicle Sensors/2 -> Behavioural Planner/1
  Behavioural Planner/1 -> Longitudinal and Lateral Controllers/1(Speed Reference)
  Behavioural Planner/2 -> Longitudinal and Lateral Controllers/2(Inter Vehicular Distance)
  Behavioural Planner/3 -> Longitudinal and Lateral Controllers/3(Lead Speed)
  Behavioural Planner/4 -> Longitudinal and Lateral Controllers/4(drivingMode)
  Behavioural Planner/5 -> Longitudinal and Lateral Controllers/5(Dist2Stop)
  Transform to MOBATSim Coordinates/1(Position) -> Position/1
  Transform to MOBATSim Coordinates/2(Orientation) -> Orientation/1
  Vehicle Model/2(Speed) -> Longitudinal and Lateral Controllers/8(Actual Speed), Speed/1
  Vehicle Model/1(Pose) -> Longitudinal and Lateral Controllers/7(Actual Pose), Transform to MOBATSim Coordinates/1(Pose)
  Longitudinal and Lateral Controllers/1(Longitudinal Acceleration Cmd) -> Vehicle Status Check and Acceleration to Speed/1(Reference Acceleration)
  Longitudinal and Lateral Controllers/2(Reference Steering Angle) -> Vehicle Status Check and Acceleration to Speed/2(Reference Steering Angle)
  Vehicle Status Check and Acceleration to Speed/2(Steering Angle Cmd) -> Vehicle Model/2(Steering Angle)
  Behavioural Planner/6 -> Longitudinal and Lateral Controllers/6(laneChange)
  Vehicle Sensors/1 -> Path Planner/1(CommunicationIDs)
  Path Planner/1(waypointReached) -> Vehicle V2I Output/1
  Vehicle Status Check and Acceleration to Speed/1(Speed Cmd) -> Vehicle Model/1(Longitudinal Speed)

== system MOBATSim/Vehicle Model 7 ==
  note: Perception
  note: Decision-Making
  note: Control
  Behavioural Planner : MATLABSystem  System=VehicleDrivingMode  Vehicle_id=Vehicle_id  SimulateUsing=Interpreted execution
      mask Type: VehicleDrivingMode
      mask Display:
      | image('MOBATSIM-Icon-Set_7- Behavioural Planner.png');
      | port_label('input',1,'vehicleDetected');
      | port_label('output',1,'SpeedReference');
      | port_label('output',2,'DistanceReference');
      | port_label('output',3,'LeadSpeed');
      | port_label('output',4,'DrivingMode');
      | port_label('output',5,'Dist2Stop');
      | port_label('output',6,'laneChange');
  Longitudinal and Lateral Controllers : Subsystem
  Path Planner : Subsystem  Variant=on  VariantControlMode=label  LabelModeActiveChoice=Astar  mask{PathPlanningAlgorithm=Astar}
      mask prompts: PathPlanningAlgorithm "Path Planning Algorithm"
      mask TypeOptions PathPlanningAlgorithm: Astar | ShortestPathFinder
      mask Callback PathPlanningAlgorithm: set_param(gcb,'OverrideUsingVariant',get_param(gcb,'PathPlanningAlgorithm'));
      mask Display: image("MOBATSIM-Icon-Set_8- Navigation.png");
  Transform to MOBATSim Coordinates : Subsystem
  Vehicle Model : Subsystem  mask{Vehicle_id=Vehicle_id}
      mask prompts: Vehicle_id "Vehicle ID"
      mask Display: image('MOBATSIM-Icon-Set_13- VehicleModel.png'); % Use "Edit Image" on toolstrip to change.
  Vehicle Sensors : MATLABSystem  System=VehicleSensors  Vehicle_id=Vehicle_id  Tsample=Sim_Ts  OffsetTime=0  SimulateUsing=Interpreted execution
      mask Type: VehicleSensors
      mask Display:
      | image('MOBATSIM-Icon-Set_4- Sensor.png');
      | port_label('output',1,'V2VcommIDs');
      | port_label('output',2,'vehicleDetected');
  Vehicle Status Check and Acceleration to Speed : Subsystem
  Vehicle V2I Output : MATLABSystem  System=VehicleV2I_Out  Vehicle_id=Vehicle_id  SimulateUsing=Interpreted execution
      mask Type: VehicleV2I_Out
      mask Display:
      | image('MOBATSIM-Icon-Set_6- V2l.png');
      | port_label('input',1,'waypointReached');
      | port_label('output',1,'V2Idata');
  Position : Outport  VectorParamsAs1DForOutWhenUnconnected=off
  Orientation : Outport  Port=2  VectorParamsAs1DForOutWhenUnconnected=off
  Speed : Outport  Port=3  VectorParamsAs1DForOutWhenUnconnected=off
  V_Network_Out : Outport  Port=4  VectorParamsAs1DForOutWhenUnconnected=off
  wires:
  Vehicle V2I Output/1 -> V_Network_Out/1
  Vehicle Sensors/2 -> Behavioural Planner/1
  Behavioural Planner/1 -> Longitudinal and Lateral Controllers/1(Speed Reference)
  Behavioural Planner/2 -> Longitudinal and Lateral Controllers/2(Inter Vehicular Distance)
  Behavioural Planner/3 -> Longitudinal and Lateral Controllers/3(Lead Speed)
  Behavioural Planner/4 -> Longitudinal and Lateral Controllers/4(drivingMode)
  Behavioural Planner/5 -> Longitudinal and Lateral Controllers/5(Dist2Stop)
  Transform to MOBATSim Coordinates/1(Position) -> Position/1
  Transform to MOBATSim Coordinates/2(Orientation) -> Orientation/1
  Vehicle Model/2(Speed) -> Longitudinal and Lateral Controllers/8(Actual Speed), Speed/1
  Vehicle Model/1(Pose) -> Longitudinal and Lateral Controllers/7(Actual Pose), Transform to MOBATSim Coordinates/1(Pose)
  Longitudinal and Lateral Controllers/1(Longitudinal Acceleration Cmd) -> Vehicle Status Check and Acceleration to Speed/1(Reference Acceleration)
  Longitudinal and Lateral Controllers/2(Reference Steering Angle) -> Vehicle Status Check and Acceleration to Speed/2(Reference Steering Angle)
  Vehicle Status Check and Acceleration to Speed/2(Steering Angle Cmd) -> Vehicle Model/2(Steering Angle)
  Behavioural Planner/6 -> Longitudinal and Lateral Controllers/6(laneChange)
  Vehicle Sensors/1 -> Path Planner/1(CommunicationIDs)
  Path Planner/1(waypointReached) -> Vehicle V2I Output/1
  Vehicle Status Check and Acceleration to Speed/1(Speed Cmd) -> Vehicle Model/1(Longitudinal Speed)

== system MOBATSim/Vehicle Model 8 ==
  note: Perception
  note: Decision-Making
  note: Control
  Behavioural Planner : MATLABSystem  System=VehicleDrivingMode  Vehicle_id=Vehicle_id  SimulateUsing=Interpreted execution
      mask Type: VehicleDrivingMode
      mask Display:
      | image('MOBATSIM-Icon-Set_7- Behavioural Planner.png');
      | port_label('input',1,'vehicleDetected');
      | port_label('output',1,'SpeedReference');
      | port_label('output',2,'DistanceReference');
      | port_label('output',3,'LeadSpeed');
      | port_label('output',4,'DrivingMode');
      | port_label('output',5,'Dist2Stop');
      | port_label('output',6,'laneChange');
  Longitudinal and Lateral Controllers : Subsystem
  Path Planner : Subsystem  Variant=on  VariantControlMode=label  LabelModeActiveChoice=Astar  mask{PathPlanningAlgorithm=Astar}
      mask prompts: PathPlanningAlgorithm "Path Planning Algorithm"
      mask TypeOptions PathPlanningAlgorithm: Astar | ShortestPathFinder
      mask Callback PathPlanningAlgorithm: set_param(gcb,'OverrideUsingVariant',get_param(gcb,'PathPlanningAlgorithm'));
      mask Display: image("MOBATSIM-Icon-Set_8- Navigation.png");
  Transform to MOBATSim Coordinates : Subsystem
  Vehicle Model : Subsystem  mask{Vehicle_id=Vehicle_id}
      mask prompts: Vehicle_id "Vehicle ID"
      mask Display: image('MOBATSIM-Icon-Set_13- VehicleModel.png'); % Use "Edit Image" on toolstrip to change.
  Vehicle Sensors : MATLABSystem  System=VehicleSensors  Vehicle_id=Vehicle_id  Tsample=Sim_Ts  OffsetTime=0  SimulateUsing=Interpreted execution
      mask Type: VehicleSensors
      mask Display:
      | image('MOBATSIM-Icon-Set_4- Sensor.png');
      | port_label('output',1,'V2VcommIDs');
      | port_label('output',2,'vehicleDetected');
  Vehicle Status Check and Acceleration to Speed : Subsystem
  Vehicle V2I Output : MATLABSystem  System=VehicleV2I_Out  Vehicle_id=Vehicle_id  SimulateUsing=Interpreted execution
      mask Type: VehicleV2I_Out
      mask Display:
      | image('MOBATSIM-Icon-Set_6- V2l.png');
      | port_label('input',1,'waypointReached');
      | port_label('output',1,'V2Idata');
  Position : Outport  VectorParamsAs1DForOutWhenUnconnected=off
  Orientation : Outport  Port=2  VectorParamsAs1DForOutWhenUnconnected=off
  Speed : Outport  Port=3  VectorParamsAs1DForOutWhenUnconnected=off
  V_Network_Out : Outport  Port=4  VectorParamsAs1DForOutWhenUnconnected=off
  wires:
  Vehicle V2I Output/1 -> V_Network_Out/1
  Vehicle Sensors/2 -> Behavioural Planner/1
  Behavioural Planner/1 -> Longitudinal and Lateral Controllers/1(Speed Reference)
  Behavioural Planner/2 -> Longitudinal and Lateral Controllers/2(Inter Vehicular Distance)
  Behavioural Planner/3 -> Longitudinal and Lateral Controllers/3(Lead Speed)
  Behavioural Planner/4 -> Longitudinal and Lateral Controllers/4(drivingMode)
  Behavioural Planner/5 -> Longitudinal and Lateral Controllers/5(Dist2Stop)
  Transform to MOBATSim Coordinates/1(Position) -> Position/1
  Transform to MOBATSim Coordinates/2(Orientation) -> Orientation/1
  Vehicle Model/2(Speed) -> Longitudinal and Lateral Controllers/8(Actual Speed), Speed/1
  Vehicle Model/1(Pose) -> Longitudinal and Lateral Controllers/7(Actual Pose), Transform to MOBATSim Coordinates/1(Pose)
  Longitudinal and Lateral Controllers/1(Longitudinal Acceleration Cmd) -> Vehicle Status Check and Acceleration to Speed/1(Reference Acceleration)
  Longitudinal and Lateral Controllers/2(Reference Steering Angle) -> Vehicle Status Check and Acceleration to Speed/2(Reference Steering Angle)
  Vehicle Status Check and Acceleration to Speed/2(Steering Angle Cmd) -> Vehicle Model/2(Steering Angle)
  Behavioural Planner/6 -> Longitudinal and Lateral Controllers/6(laneChange)
  Vehicle Sensors/1 -> Path Planner/1(CommunicationIDs)
  Path Planner/1(waypointReached) -> Vehicle V2I Output/1
  Vehicle Status Check and Acceleration to Speed/1(Speed Cmd) -> Vehicle Model/1(Longitudinal Speed)
